simulink model "arducopter"  (R2024b)
settings: Solver=FixedStepAuto  StartTime=0.0  StopTime=simIn.param.timeEnd  FixedStep=simIn.param.dt  RelTol=1e-3
undefined symbols (not defined in the file or in its folder): DiscIntNeverNeededParam, sim, simIn
libraries: simulink x60, slident x4, vrlib x1
(part 1 of 9)
settings Model: Creator=f02brede  LastModifiedBy=I012407
settings SolverCC: AlgebraicLoopSolver=TrustRegion
settings OptimizationCC: BlockReduction=off  DefaultParameterBehavior=Inlined  BufferReuse=off
settings DebuggingCC: ParamSuppressDoubleToSinglePrecisionLossMsg=on  UnconnectedInputMsg=warning  UnconnectedOutputMsg=warning  UnconnectedLineMsg=warning  UnderSpecifiedDimensionMsg=warning
settings ModelReferenceCC: EnableRefExpFcnMdlSchedulingChecks=on
settings RTWCC: GPUComputeCapability=3.5  DLArmComputeVersion=19.05

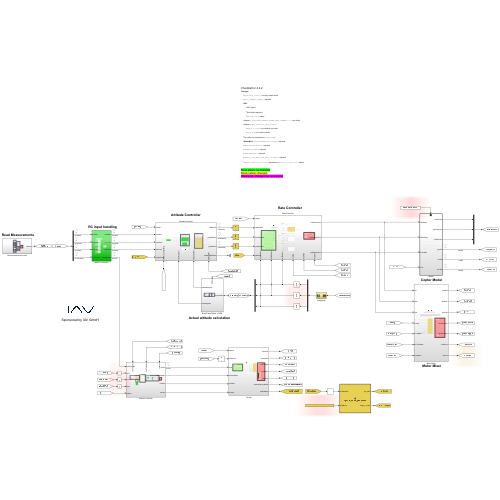
[thumbnail: Simulink's stored preview of the top-level diagram]
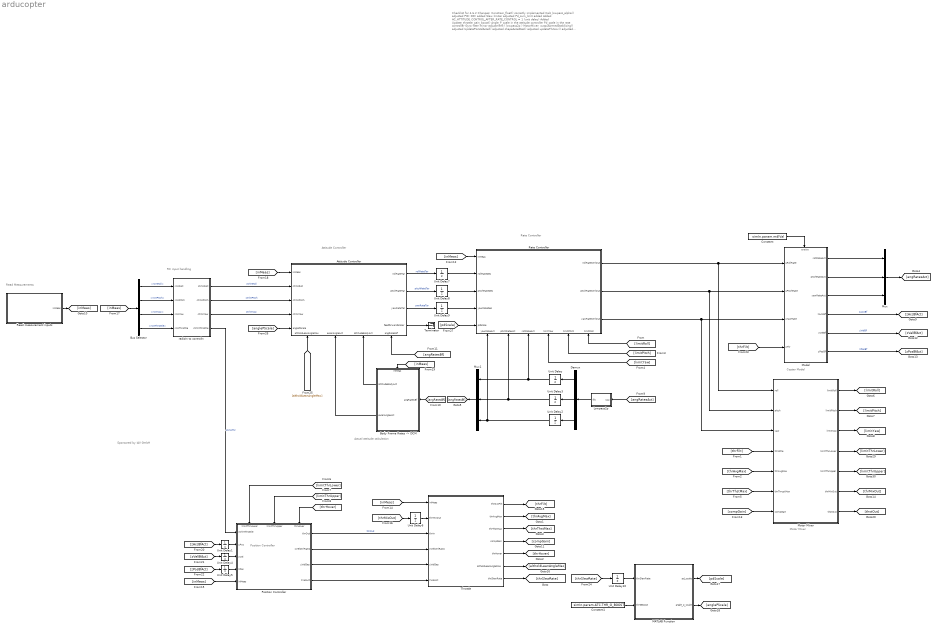
== system arducopter ==
  note: Checklist for 4.6.2
      | Changes:
      | Constrain_float() correctly implemented
      | Calc_lowpass_alpha() adjusted
      | PID: DFF added
      | Slew limiter adjusted
      | Pd_sum_limit added
      |
      | Added AC_ATTITUDE_CONTROL_AFTER_RATE_CONTROL = 1 (unit delay)
      | Added Update_throttle_gain_boost() Angle_P_scale in the attitude controller
      | Pd_scale in the rate controller
      |
      | Gyro filter minor adjustment ( lowpass2p )
      | MotorMixer: outputArmedStabilizing() adjusted
      | UpdatePosVelAccel() adjusted
      | shapeAccelDes() adjusted
      | updateThrHov() adjusted
      | Update_lift_max_from_batt_voltage() adjusted
      | Update_throttle_filter() adjusted and throttle_slew_filter added
      |
      | Bock green: no changes
      | Block yellow: changes
      | Block pink: changes but no solution
  note: Read Measurements
  note: RC input handling
  note: Attitude Controller
  note: Position Controller
  note: Actual attitude calculation
  note: Rate Controller
  note: Copter Model
  note: Motor Mixer
  note: Sponsored by IAV GmbH
  Attitude Controller : Subsystem
      settings: PortSchema="{\"entries\":[{\"content\":{\"sides\":[{\"content\":{\"connectorIds\":[\"In1\",\"In2\",\"In3\",\"In4\",\"In5\"]},\"type\":\"ConnectorPlacement.EquallySpacedRectSide\",\"uuid\":\"be329309-f60f-4247-8f12-99293f1f15e2\"},{\"content\":{\"connectorIds\":[\"Out1\",\"Out2\",\"Out3\",\"Out4\"],\"side\":\"RIGHT\"},\"type\":\"ConnectorPlacement.EquallySpacedRectSide\",\"uuid\":\"c2d00d61-d122-496e-b903-ccd22f2a218f\"},{\"content\":{\"side\":\"TOP\"},\"type\":\"ConnectorPlacement.EquallySpacedRectSide\",\"uuid\":\"754e14e5-9744-47de-9a4b-82f23abee3a3\"},{\"content\":{\"connectorIds\":[\"In6\",\"In7\",\"In8\",\"In9\"],\"side\":\"BOTTOM\"},\"type\":\"ConnectorPlacement.EquallySpacedRectSide\",\"uuid\":\"be89750d-8e93-4dd5-898c-e5776ff84547\"}]},\"type\":\"ConnectorPlacement.EquallySpacedConnector\",\"uuid\":\"7867ed09-773f-4285-9280-958eb598c3c9\"}],\"packageUris\":[\"http://schema.mathworks.com/mf0/Connector/R2020b\"],\"version\":\"1.0\"}"
  "Body Frame Rates -> DCM" : Subsystem
      settings: PortSchema="{\"entries\":[{\"content\":{\"sides\":[{\"content\":{\"connectorIds\":[\"In1\"]},\"type\":\"ConnectorPlacement.EquallySpacedRectSide\",\"uuid\":\"b5a1df0d-dabf-40be-945b-766674ab7f8a\"},{\"content\":{\"connectorIds\":[\"Out1\",\"Out2\"],\"side\":\"RIGHT\"},\"type\":\"ConnectorPlacement.EquallySpacedRectSide\",\"uuid\":\"df9d5bb2-532d-49d7-bb71-db77180d8edc\"},{\"content\":{\"connectorIds\":[\"In2\"],\"side\":\"TOP\"},\"type\":\"ConnectorPlacement.EquallySpacedRectSide\",\"uuid\":\"d376726d-d96e-422a-81b7-0e4338bb2c38\"}]},\"type\":\"ConnectorPlacement.EquallySpacedConnector\",\"uuid\":\"2a47101d-f111-46e9-ab13-8c5a8aa6bb71\"}],\"packageUris\":[\"http://schema.mathworks.com/mf0/Connector/R2020b\"],\"version\":\"1.0\"}"
  Bus Selector : BusSelector  OutputSignals=RCIN.rcinRoll,RCIN.rcinPitch,RCIN.rcinYaw,RCIN.rcinThrottle
  Constant : Constant  Value=simIn.param.mdlVal
  Constant1 : Constant  Value=simIn.param.ATC.THR_G_BOOST
  Demux : Demux  Outputs=3
  Lowpass2p : Subsystem
  MATLAB Function : MATLAB Function  TreatAsAtomicUnit=on
  Model : Subsystem
  Motor Mixer : Subsystem
  Mux : Mux  Inputs=3
  Mux1 : Mux  Inputs=3
  Position Controller : Subsystem
      settings: PortSchema="{\"entries\":[{\"content\":{\"sides\":[{\"content\":{\"connectorIds\":[\"In1\",\"In2\",\"In3\",\"In4\",\"In5\"]},\"type\":\"ConnectorPlacement.EquallySpacedRectSide\",\"uuid\":\"373ae21e-4a6c-4b99-84f1-ac5f8a8ac7e4\"},{\"content\":{\"connectorIds\":[\"Out1\",\"Out2\",\"Out3\",\"Out4\"],\"side\":\"RIGHT\"},\"type\":\"ConnectorPlacement.EquallySpacedRectSide\",\"uuid\":\"b87000f3-0870-478f-96d5-bf9fbf48201f\"},{\"content\":{\"connectorIds\":[\"In6\",\"In7\",\"In8\"],\"side\":\"TOP\"},\"type\":\"ConnectorPlacement.EquallySpacedRectSide\",\"uuid\":\"fdc4322a-c616-417b-b4c1-4fa4efa7a345\"}]},\"type\":\"ConnectorPlacement.EquallySpacedConnector\",\"uuid\":\"66c5051f-cbed-470e-8eb0-2aea9e9650fc\"}],\"packageUris\":[\"http://schema.mathworks.com/mf0/Connector/R2020b\"],\"version\":\"1.0\"}"
  Rate Controller : Subsystem
      settings: PortSchema="{\"entries\":[{\"content\":{\"sides\":[{\"content\":{\"connectorIds\":[\"In1\",\"In2\",\"In3\",\"In4\",\"In5\"]},\"type\":\"ConnectorPlacement.EquallySpacedRectSide\",\"uuid\":\"8a701ca7-ce38-496e-9f89-73a8426d5a34\"},{\"content\":{\"connectorIds\":[\"Out1\",\"Out2\",\"Out3\"],\"side\":\"RIGHT\"},\"type\":\"ConnectorPlacement.EquallySpacedRectSide\",\"uuid\":\"363a0e2e-6acc-4f21-9121-ba7c8748d9b4\"},{\"content\":{\"side\":\"TOP\"},\"type\":\"ConnectorPlacement.EquallySpacedRectSide\",\"uuid\":\"4d7a2121-90ee-4dbe-91e3-b86ad0b96fd9\"},{\"content\":{\"connectorIds\":[\"In6\",\"In7\",\"In8\",\"In9\",\"In10\",\"In11\"],\"side\":\"BOTTOM\"},\"type\":\"ConnectorPlacement.EquallySpacedRectSide\",\"uuid\":\"495eef18-c57e-4f49-baa4-5500712935f3\"}]},\"type\":\"ConnectorPlacement.EquallySpacedConnector\",\"uuid\":\"9c8722b4-18d5-4647-94e4-af7446d3f664\"}],\"packageUris\":[\"http://schema.mathworks.com/mf0/Connector/R2020b\"],\"version\":\"1.0\"}"
  Read measurement inputs : Subsystem
  Terminator : Terminator
  Throttle : Subsystem
  Unit Delay{,2,6..10} (7 alike) : UnitDelay  SampleTime=-1  HasFrameUpgradeWarning=on
  Unit Delay1 : UnitDelay  InitialCondition=simIn.init.PSCD.accAct  SampleTime=-1  HasFrameUpgradeWarning=on
  Unit Delay3 : UnitDelay  InitialCondition=simIn.models.PitchInit  SampleTime=-1  HasFrameUpgradeWarning=on
  Unit Delay4 : UnitDelay  InitialCondition=simIn.init.PSCD.velAct  SampleTime=-1  HasFrameUpgradeWarning=on
  Unit Delay5 : UnitDelay  InitialCondition=simIn.init.PSCD.posAct  SampleTime=-1  HasFrameUpgradeWarning=on
  radioIn to controlIn : Subsystem
  wires:
  [compGain] -> Motor Mixer/7(compGain)
  Rate Controller/3(yawRateCtrlOut) -> Model/3(uYawRate), Motor Mixer/3(yaw)
  Motor Mixer/5(limitThrUpper) -> [limitThrUpper]
  [thrThstMax] -> Motor Mixer/6(thrThrustMax)
  Motor Mixer/4(limitThrLower) -> [limitThrLower]
  Motor Mixer/7(thstOut) -> [thstOut]
  Motor Mixer/2(limitPitch) -> [limitPitch]
  Motor Mixer/3(limitYaw) -> [limitYaw]
  Motor Mixer/6(thrMixOut) -> [thrMixOut]
  [thrFilt] -> Motor Mixer/4(throttle)
  [thrAvgMax] -> Motor Mixer/5(thrAvgMax)
  Motor Mixer/1(limitRoll) -> [limitRoll]
  Throttle/2(thrAvgMax) -> [thrAvgMax]
  Throttle/3(thrThstMax) -> [thrThstMax]
  Throttle/4(compGain) -> [compGain]
  [limitYaw] -> Rate Controller/9(limitYaw)
  [limitPitch] -> Rate Controller/10(limitPitch)
  [limitRoll] -> Rate Controller/11(limitRoll)
  Throttle/5(thrHover) -> [thrHover]
  [limitThrLower] -> Position Controller/6(limitThrLower)
  [limitThrUpper] -> Position Controller/7(limitThrUpper)
  Position Controller/1(thrOut) -> Throttle/3(thrIn)  "thrOut"
  Position Controller/2(zVelCtrlRatio) -> Throttle/4(zVelCtrlRatio)
  Position Controller/3(zVelDes) -> Throttle/5(zVelDes)
  Position Controller/4(zVelAct) -> Throttle/6(zVelAct)
  Model/1(rollRateAct) -> Mux/1
  Model/2(pitchRateAct) -> Mux/2
  Model/3(yawRateAct) -> Mux/3
  Unit Delay/1 -> Mux1/1, Rate Controller/8(rollRateAct)
  Unit Delay2/1 -> Mux1/3, Rate Controller/6(yawRateAct)
  Read measurement inputs/1(inMeas) -> [inMeas]
  [inMeas] -> Rate Controller/1(inMeas)
  [inMeas] -> Throttle/1(inMeas)
  [inMeas] -> Position Controller/5(inMeas)
  [inMeas] -> Bus Selector/1
  Demux/2 -> Unit Delay3/1
  Mux/1 -> [angRatesAct]
  Demux/1 -> Unit Delay/1
  Demux/3 -> Unit Delay2/1
  [angRatesAct] -> Lowpass2p/1(raw)
  Lowpass2p/1(filt) -> Demux/1
  Unit Delay3/1 -> Mux1/2, Rate Controller/7(pitchRateAct)
  Rate Controller/2(pitchRateCtrlOut) -> Motor Mixer/2(pitch), Model/2(uPitchRate)
  Rate Controller/1(rollRateCtrlOut) -> Motor Mixer/1(roll), Model/1(uRollRate)
  Attitude Controller/2(pitchRateTar) -> Unit Delay8/1  "pitchRateTar"
  Attitude Controller/3(yawRateTar) -> Unit Delay9/1  "yawRateTar"
  Bus Selector/1 -> radioIn to controlIn/1(rcInRoll)  "<rcinRoll>"
  Bus Selector/2 -> radioIn to controlIn/2(rcInPitch)  "<rcinPitch>"
  Bus Selector/3 -> radioIn to controlIn/3(rcInYaw)  "<rcinYaw>"
  "Body Frame Rates -> DCM"/1(attitudeBodyAct) -> Attitude Controller/8(attitudeBodyAct)
  Mux1/1 -> [angRatesBf]
  [angRatesBf] -> "Body Frame Rates -> DCM"/1(angRatesBf)
  [angRatesBf] -> Attitude Controller/9(angRatesBf)
  [inMeas] -> Attitude Controller/1(inMeas)
  Attitude Controller/4(feedforwardScaler) -> Terminator/1
  [inMeas] -> "Body Frame Rates -> DCM"/2(inMeas)
  radioIn to controlIn/1(ctrlInRoll) -> Attitude Controller/2(ctrlInRoll)  "ctrlInRoll"
  radioIn to controlIn/2(ctrlInPitch) -> Attitude Controller/3(ctrlInPitch)  "ctrlInPitch"
  radioIn to controlIn/3(ctrlInYaw) -> Attitude Controller/4(ctrlInYaw)  "ctrlInYaw"
  Attitude Controller/1(rollRateTar) -> Unit Delay7/1  "rollRateTar"
  Constant/1 -> Model/Enable
  "Body Frame Rates -> DCM"/2(eulerAngleAct) -> Attitude Controller/7(eulerAngleAct)
  Model/4(zAccBf) -> [zAccBfAct]  "zAccBf"
  [thrFilt] -> Model/4(uThr)
  Model/5(zVelBf) -> [zVelBfAct]  "zVelBf"
  Model/6(zPosBf) -> [zPosBfAct]  "zPosBf"
  [zAccBfAct] -> Unit Delay1/1
  [zVelBfAct] -> Unit Delay4/1
  [zPosBfAct] -> Unit Delay5/1
  [thrHover] -> Position Controller/8(thrHover)
  Unit Delay1/1 -> Position Controller/2(zAcc)
  Unit Delay4/1 -> Position Controller/3(zVel)
  Unit Delay5/1 -> Position Controller/4(zPos)
  Bus Selector/4 -> radioIn to controlIn/4(rcInThrottle)  "<rcinThrottle>"
  radioIn to controlIn/4(ctrlInThrottle) -> Position Controller/1(ctrlInThrottle)  "ctrlInThr"
  Throttle/1(thrOutFilt) -> [thrFilt]
  [thrMixOut] -> Unit Delay6/1
  Unit Delay6/1 -> Throttle/2(thrMixOut)
  [altholdLeanAngleMax] -> Attitude Controller/6(altholdLeanAngleMax)
  Throttle/6(altholdLeanAngleMax) -> [altholdLeanAngleMax]
  Unit Delay9/1 -> Rate Controller/4(yawRateDes)
  Unit Delay8/1 -> Rate Controller/3(pitchRateDes)
  Unit Delay7/1 -> Rate Controller/2(rollRateDes)
  Throttle/7(thrSlewRate) -> [thrSlewRate]
  Constant1/1 -> MATLAB Function/2(thrGBoost)
  [thrSlewRate] -> Unit Delay10/1
  MATLAB Function/1(pd_scale) -> [pdScale]
  MATLAB Function/2(angle_p_scale) -> [anglePScale]
  [anglePScale] -> Attitude Controller/5(anglePScale)
  [pdScale] -> Rate Controller/5(pdScale)
  Unit Delay10/1 -> MATLAB Function/1(thrSlewRate)

== system arducopter/Attitude Controller ==
  note: input_euler_angle_roll_pitch_euler_rate_yaw() & attitude_controller_run_quat()
      | Calculation of target euler rates and angles and angular velocities
  note: Mode::get_pilot_desired_lean_angles() & Mode::get_pilot_desired_yaw_rate()
      | Conversion from raw pilot inputs to desired roll and pitch angles and yaw rate
  note: Determines the angleLimit (angle_limit_cd) based on the flight mode
  note: Sponsored by IAV GmbH
  inMeas : Inport
  ctrlInRoll : Inport  Port=2
  ctrlInPitch : Inport  Port=3
  ctrlInYaw : Inport  Port=4
  anglePScale : Inport  Port=5
  altholdLeanAngleMax : Inport  Port=6
  eulerAngleAct : Inport  Port=7
  attitudeBodyAct : Inport  Port=8
  angRatesBf : Inport  Port=9
  Bus Selector : BusSelector  OutputSignals=CTUN.thrInMeas
  Constant : Constant  Value=simIn.param.ANGLE_MAX
  Constant1 : Constant  Value=simIn.param.PILOT_Y_EXPO
  Constant2 : Constant  Value=simIn.param.PILOT_Y_RATE
  Constant3 : Constant  Value=simIn.param.RCIN.ROLL_PITCH_YAW_INPUT_MAX
  Demux : Demux  Outputs=3
  Determine angleLimit : Subsystem
  MATLAB Function : MATLAB Function  TreatAsAtomicUnit=on
  MATLAB Function1 : MATLAB Function  TreatAsAtomicUnit=on
  cdeg to radians : Gain  Gain=0.01*pi/180
  cdeg to radians1 : Gain  Gain=0.01*pi/180
  cdeg/s to radians/s : Gain  Gain=0.01*pi/180
  input_euler_angle_roll_pitch_euler_rate_yaw() : Subsystem
      settings: PortSchema="{\"entries\":[{\"content\":{\"sides\":[{\"content\":{\"connectorIds\":[\"In1\",\"In2\",\"In3\",\"In4\",\"In5\",\"In6\"]},\"type\":\"ConnectorPlacement.EquallySpacedRectSide\",\"uuid\":\"a7f2758f-6981-4691-a616-9de398d31e49\"},{\"content\":{\"connectorIds\":[\"Out1\",\"Out2\"],\"side\":\"RIGHT\"},\"type\":\"ConnectorPlacement.EquallySpacedRectSide\",\"uuid\":\"ab82c46a-21a0-4466-8d5f-7cb35c1d2ba7\"},{\"content\":{\"connectorIds\":[\"In7\",\"In8\"],\"side\":\"TOP\"},\"type\":\"ConnectorPlacement.EquallySpacedRectSide\",\"uuid\":\"f47afcce-c5f7-4588-aa52-961f89e87fe1\"}]},\"type\":\"ConnectorPlacement.EquallySpacedConnector\",\"uuid\":\"c65a3016-6632-4380-919e-0448495ac13d\"}],\"packageUris\":[\"http://schema.mathworks.com/mf0/Connector/R2020b\"],\"version\":\"1.0\"}"
  rollRateTar : Outport
  pitchRateTar : Outport  Port=2
  yawRateTar : Outport  Port=3
  feedforwardScaler : Outport  Port=4
  wires:
  ctrlInRoll/1 -> MATLAB Function/1(rollIn)
  ctrlInPitch/1 -> MATLAB Function/2(pitchIn)
  Constant/1 -> MATLAB Function/3(angleMax)
  Constant1/1 -> MATLAB Function1/2(pilotYawExpo)
  Constant2/1 -> MATLAB Function1/3(pilotYawRate)
  MATLAB Function/1(rollOut) -> cdeg to radians/1
  MATLAB Function/2(pitchOut) -> cdeg to radians1/1
  cdeg to radians/1 -> input_euler_angle_roll_pitch_euler_rate_yaw()/1(rollAngDes)  "rollLeanAngleDes"
  cdeg to radians1/1 -> input_euler_angle_roll_pitch_euler_rate_yaw()/2(pitchAngDes)  "pitchLeanAngleDes"
  attitudeBodyAct/1 -> input_euler_angle_roll_pitch_euler_rate_yaw()/5(attitudeBodyAct)
  angRatesBf/1 -> input_euler_angle_roll_pitch_euler_rate_yaw()/6(angRatesBf)
  Demux/2 -> pitchRateTar/1
  Demux/1 -> rollRateTar/1
  Demux/3 -> yawRateTar/1
  input_euler_angle_roll_pitch_euler_rate_yaw()/1(angVelBodyTarget) -> Demux/1  "angVelBody"
  input_euler_angle_roll_pitch_euler_rate_yaw()/2(feedforwardScaler) -> feedforwardScaler/1
  inMeas/1 -> Bus Selector/1
  Bus Selector/1 -> [throttle]  "<thrInMeas>"
  [throttle] -> input_euler_angle_roll_pitch_euler_rate_yaw()/7(throttle)
  eulerAngleAct/1 -> input_euler_angle_roll_pitch_euler_rate_yaw()/4(eulerAngleAct)
  ctrlInYaw/1 -> MATLAB Function1/1(yawIn)
  Constant3/1 -> MATLAB Function/5(rpyInputMax)
  cdeg/s to radians/s/1 -> input_euler_angle_roll_pitch_euler_rate_yaw()/3(yawRateDes)  "yawRateDes"
  MATLAB Function1/1(yawOut) -> cdeg/s to radians/s/1  "yawRateDes"
  altholdLeanAngleMax/1 -> Determine angleLimit/1(altholdLeanAngleMax)
  Determine angleLimit/1(angleLimit) -> MATLAB Function/4(angleLimit)
  anglePScale/1 -> input_euler_angle_roll_pitch_euler_rate_yaw()/8(anglePScale)

== system arducopter/Body Frame Rates -> DCM ==
  note: QuaternionT<T>::from_rotation_matrix()
      | Calculation of the quaternion of the body-frame attitude.
      | Function is called in AC_AttitudeControl::attitude_controller_run_quat() -> AP_AHRS::get_quat_body_to_ned()
  note: The resulting matrix is updated in AP_AHRS_View::update(). There, it is rotated by the rotation matrix of the view, which is created in the constructor of AP_AHRS_View. For a copter, it is zero (see system.cpp: ahrs_view = ahrs.create_view(ROTATION_NONE))
      |
      | The resulting matrix represents the rotation matrix that is used to calculate the "measured" angles of the ATT message.
  note: $\Delta \underline{\underline{R}} = \underline{\underline{R}} \, \Delta \underline{\underline{w}}$
  note: Taken from Matrix3<T>::rotate() in matrix.cpp
  note: Source: https://academicflight.com/articles/kinematics/rotation-formalisms/rotation-matrix/
  note: Create cross-product equivalent matrix of vector
  note: Source: AP_AHRS_DCM::matrix_update() and Matrix3<T>::rotate()
      | - Corrections for gyro drifts (_omega_I, _omega_P, _omega_yaw_P) were left out.
  note: Update DCM matrix
  note: $\Delta \underline{\underline{w}} = \underline{\underline{\omega}} \, T_s$
  note: $\underline{\underline{R}}_{\, \mathrm{k}} = \Delta \underline{\underline{R}} + \underline{\underline{R}}_{\, \mathrm{k-1}}$
  note: Calculation of _body_dcm_matrix aka rot_body_to_ned
  note: Correction of DCM by difference between controller and body
      | frames.
      | Taken from AP_AHRS_DCM::euler_angles()
  note: Sponsored by IAV GmbH
  angRatesBf : Inport
  inMeas : Inport  Port=2
  BF2FC : Constant  Value=simIn.param.AHRS.BF2FC
  Bus Selector : BusSelector  OutputSignals=ATT.rollAngleActMeas,ATT.pitchAngleActMeas,ATT.yawAngleActMeas
  Bus Selector1 : BusSelector  OutputSignals=ATT.rollAngleActMeas,ATT.pitchAngleActMeas,ATT.yawAngleActMeas
  Constant : Constant  Value=0  OutDataTypeStr=single
  Constant1 : Constant  Value=simIn.param.attCtrlVal
  Constant4 : Constant  Value=simIn.param.attCtrlVal
  Data Type Conversion : DataTypeConversion  OutDataTypeStr=single  SaturateOnIntegerOverflow=off  RndMeth=Floor
  Data Type Conversion1 : DataTypeConversion  OutDataTypeStr=single  SaturateOnIntegerOverflow=off  RndMeth=Floor
  Gain2 : Gain  Gain=simIn.param.dt  OutDataTypeStr=single
  Gain3 : Gain  Gain=[1 1 -1]
  Gain4 : Gain  Gain=[-1 1 1]
  Gain5 : Gain  Gain=[1 -1 1]
  MATLAB Function : MATLAB Function  TreatAsAtomicUnit=on
  MATLAB Function1 : MATLAB Function  TreatAsAtomicUnit=on
  MATLAB Function2 : MATLAB Function  TreatAsAtomicUnit=on
  MATLAB Function3 : MATLAB Function  TreatAsAtomicUnit=on
  Matrix Concatenate : Concatenate  NumInputs=3  Mode=Multidimensional array  ConcatenateDimension=2
  Mux : Mux  Inputs=3
  Mux1 : Mux  Inputs=3
  Product : Product  Multiplication=Matrix(*)
  Product1 : Product  Multiplication=Matrix(*)
  Selector : Selector  InputPortWidth=4  IndexOptions=Index vector (dialog)  Indices=[1 4 3]  OutputSizes=1
  Selector1 : Selector  InputPortWidth=4  IndexOptions=Index vector (dialog)  Indices=[4 1 2]  OutputSizes=1
  Selector2 : Selector  InputPortWidth=4  IndexOptions=Index vector (dialog)  Indices=[3 2 1]  OutputSizes=1
  Sum : Sum  Inputs=++|
  Switch : Switch  Criteria=u2 > Threshold  SaturateOnIntegerOverflow=off  InputSameDT=off
  Switch1 : Switch  Criteria=u2 > Threshold  SaturateOnIntegerOverflow=off  InputSameDT=off
  Unit Delay : UnitDelay  InitialCondition=simIn.init.ATT.DCM  SampleTime=-1  HasFrameUpgradeWarning=on
  Vector Concatenate : Concatenate
  attitudeBodyAct : Outport
  eulerAngleAct : Outport  Port=2
  wires:
  angRatesBf/1 -> Vector Concatenate/2
  Vector Concatenate/1 -> Selector/1, Selector1/1, Selector2/1
  Selector/1 -> Gain3/1
  Constant/1 -> Vector Concatenate/1
  Selector2/1 -> Gain5/1
  Selector1/1 -> Gain4/1
  Gain3/1 -> Matrix Concatenate/1
  Gain4/1 -> Matrix Concatenate/2
  Gain5/1 -> Matrix Concatenate/3
  Matrix Concatenate/1 -> Gain2/1
  Unit Delay/1 -> Product/1, Sum/1
  Product/1 -> Sum/2
  Sum/1 -> Product1/1, Unit Delay/1  "DCM"
  Gain2/1 -> Product/2
  BF2FC/1 -> Product1/2
  Product1/1 -> MATLAB Function1/1(rotMat), MATLAB Function/1(dcm)  "bodyDCM"
  MATLAB Function/1(quaternion) -> Data Type Conversion/1
  [meas] -> Bus Selector/1
  Bus Selector/2 -> MATLAB Function2/2(pitch)  "<pitchAngleActMeas>"
  Bus Selector/1 -> MATLAB Function2/1(roll)  "<rollAngleActMeas>"
  Bus Selector/3 -> MATLAB Function2/3(yaw)  "<yawAngleActMeas>"
  MATLAB Function3/1(quaternion) -> Data Type Conversion1/1
  MATLAB Function2/1(rotMat) -> MATLAB Function3/1(dcm)  "bodyDCMMeas"
  MATLAB Function1/1(roll) -> Mux/1  "rollAngleAct"
  MATLAB Function1/2(pitch) -> Mux/2  "pitchAngleAct"
  MATLAB Function1/3(yaw) -> Mux/3  "yawAngleAct"
  Switch/1 -> attitudeBodyAct/1
  Data Type Conversion1/1 -> Switch/1
  Data Type Conversion/1 -> Switch/3
  Constant4/1 -> Switch/2
  Switch1/1 -> eulerAngleAct/1
  Constant1/1 -> Switch1/2
  Mux/1 -> Switch1/3
  inMeas/1 -> [meas]
  [meas] -> Bus Selector1/1
  Bus Selector1/1 -> Mux1/1  "<rollAngleActMeas>"
  Bus Selector1/2 -> Mux1/2  "<pitchAngleActMeas>"
  Bus Selector1/3 -> Mux1/3  "<yawAngleActMeas>"
  Mux1/1 -> Switch1/1

== system arducopter/Lowpass2p ==
  raw : Inport
  Constant : Constant  Value=simIn.param.INS.GYRO_FILTER
  Constant1 : Constant  Value=simIn.param.INS.GYRO_RATE
  Demux : Demux  Outputs=3
  Lowpass Pitch : Subsystem
  Lowpass Roll : Subsystem
  Lowpass Yaw : Subsystem
  Mux : Mux  Inputs=3
  filt : Outport
  wires:
  raw/1 -> Demux/1
  Demux/1 -> [rollRaw]
  Demux/3 -> [yawRaw]
  Demux/2 -> [pitchRaw]
  [rollRaw] -> Lowpass Roll/1(sample)
  [pitchRaw] -> Lowpass Pitch/1(sample)
  [yawRaw] -> Lowpass Yaw/1(sample)
  Mux/1 -> filt/1
  Lowpass Roll/1(y) -> [rollFilt]
  Lowpass Pitch/1(y) -> [pitchFilt]
  Lowpass Yaw/1(y) -> [yawFilt]
  [rollFilt] -> Mux/1
  [pitchFilt] -> Mux/2
  [yawFilt] -> Mux/3
  Constant/1 -> [cutoffFreq]
  Constant1/1 -> [sampleFreq]
  [sampleFreq] -> Lowpass Roll/2(sampleFreq)
  [cutoffFreq] -> Lowpass Roll/3(cutoffFreq)
  [cutoffFreq] -> Lowpass Pitch/3(cutoffFreq)
  [sampleFreq] -> Lowpass Pitch/2(sampleFreq)
  [sampleFreq] -> Lowpass Yaw/2(sampleFreq)
  [cutoffFreq] -> Lowpass Yaw/3(cutoffFreq)

== system arducopter/Model ==
  uRollRate : Inport
  uPitchRate : Inport  Port=2
  uYawRate : Inport  Port=3
  uThr : Inport  Port=4
  Enable : EnablePort
  Constant : Constant  Value=simIn.models.VerticalInInit
  Data Type Conversion{,2..3,6} (4 alike) : DataTypeConversion  OutDataTypeStr=double  SaturateOnIntegerOverflow=off  RndMeth=Floor
  Data Type Conversion{1,4..5,7} (4 alike) : DataTypeConversion  OutDataTypeStr=single  SaturateOnIntegerOverflow=off  RndMeth=Floor
  Discrete-Time Integrator : DiscreteIntegrator  InitialCondition=simIn.init.PSCD.velAct  SampleTime=0.0025  ICPrevOutput=DiscIntNeverNeededParam  ICPrevScaledInput=DiscIntNeverNeededParam
  Discrete-Time Integrator1 : DiscreteIntegrator  InitialCondition=simIn.init.PSCD.posAct  SampleTime=-1  ICPrevOutput=DiscIntNeverNeededParam  ICPrevScaledInput=DiscIntNeverNeededParam
  Idmodel : slident/Models/Idmodel  sys=simIn.models.PitchAxis  IC=simIn.models.PitchInit  noi=off  seed=[]
  Idmodel1 : slident/Models/Idmodel  sys=simIn.models.RollAxis  IC=simIn.models.RollInit  noi=off  seed=[]
  Idmodel2 : slident/Models/Idmodel  sys=simIn.models.YawAxis  IC=simIn.models.YawInit  noi=off  seed=[]
  Idmodel3 : slident/Models/Idmodel  sys=simIn.models.VerticalAxis  IC=0  noi=off  seed=[]
  Sum : Sum  Inputs=|+-
  rollRateAct : Outport
  pitchRateAct : Outport  Port=2
  yawRateAct : Outport  Port=3
  zAccBf : Outport  Port=4
  zVelBf : Outport  Port=5
  zPosBf : Outport  Port=6
  wires:
  uPitchRate/1 -> Data Type Conversion/1
  uYawRate/1 -> Data Type Conversion2/1
  Idmodel1/1 -> Data Type Conversion4/1
  uRollRate/1 -> Data Type Conversion3/1
  Idmodel2/1 -> Data Type Conversion5/1
  Data Type Conversion/1 -> Idmodel/1
  Data Type Conversion2/1 -> Idmodel2/1
  Data Type Conversion3/1 -> Idmodel1/1
  Data Type Conversion4/1 -> rollRateAct/1
  Data Type Conversion1/1 -> pitchRateAct/1
  Data Type Conversion5/1 -> yawRateAct/1
  Idmodel/1 -> Data Type Conversion1/1
  Data Type Conversion6/1 -> Idmodel3/1
  Idmodel3/1 -> Data Type Conversion7/1
  Sum/1 -> Data Type Conversion6/1
  uThr/1 -> Sum/1
  Data Type Conversion7/1 -> Discrete-Time Integrator/1, zAccBf/1
  Constant/1 -> Sum/2
  Discrete-Time Integrator/1 -> Discrete-Time Integrator1/1, zVelBf/1
  Discrete-Time Integrator1/1 -> zPosBf/1

== system arducopter/Motor Mixer ==
  note: Motor Mixer Output
  note: This function calculates the outputs to the motors based on the requested roll, pitch, yaw and throttle thrust. At first, the maximum allowed yaw is calculated. On the basis of the difference between the maximum and minimum value of the combined roll, pitch and yaw thrust of the motors, the thrust values are scaled within the valid output range. The final motor commands are calculated by the sum of the combined roll, pitch and yaw thrust and and the demanded throttle thrust, which might be set to a lower value when the combined thrust demand of roll, pitch and yaw exceed the possbile thrust.
  note: Motor Mixer - Calculation of outputs to motors.
  note: Sponsored by IAV GmbH
  roll : Inport
  pitch : Inport  Port=2
  yaw : Inport  Port=3
  throttle : Inport  Port=4
  thrAvgMax : Inport  Port=5
  thrThrustMax : Inport  Port=6
  compGain : Inport  Port=7
  Calculate motor thrust : MATLAB Function  TreatAsAtomicUnit=on
  Clock : Clock
  Constant : Constant  Value=simIn.param.NUM_MOTORS
  Constant1 : Constant  Value=simIn.param.AXIS_FAC_MOTORS.pitch  VectorParams1D=off
  Constant11 : Constant  Value=simIn.param.MOT.YAW_HEADROOM
  Constant12 : Constant  Value=simIn.param.AXIS_FAC_MOTORS.throttle  VectorParams1D=off
  Constant2 : Constant  Value=simIn.param.AXIS_FAC_MOTORS.roll  VectorParams1D=off
  Constant3 : Constant  Value=simIn.param.AXIS_FAC_MOTORS.yaw  VectorParams1D=off
  Data Store Memory : DataStoreMemory  DataStoreName=thst_rpyt  ReadBeforeWriteMsg=warning  WriteAfterWriteMsg=warning  WriteAfterReadMsg=warning  InitialValue=zeros(simIn.param.NUM_MOTORS,1)  ShowAdditionalParam=off  OutDataTypeStr=single
  Data Type Conversion1 : DataTypeConversion  OutDataTypeStr=single  SaturateOnIntegerOverflow=off  RndMeth=Floor
  Data Type Conversion2 : DataTypeConversion  OutDataTypeStr=single  SaturateOnIntegerOverflow=off  RndMeth=Floor
  Terminator6 : Terminator
  ThrMixOutMeas : Lookup_n-D  NumberOfTableDimensions=1  BreakpointsForDimension1=simIn.signals.MOTQ.Time  Table=simIn.signals.MOTQ.ThrMixOut  InternalRulePriority=Speed  RndMeth=Simplest
  Vector Concatenate : Concatenate  NumInputs=4  Mode=Multidimensional array
  limitRoll : Outport
  limitPitch : Outport  Port=2
  limitYaw : Outport  Port=3
  limitThrLower : Outport  Port=4  SampleTime=simIn.param.dt
  limitThrUpper : Outport  Port=5  SampleTime=simIn.param.dt
  thrMixOut : Outport  Port=6
  thstOut : Outport  Port=7  SampleTime=simIn.param.dt
  wires:
  roll/1 -> Calculate motor thrust/1(roll)
  throttle/1 -> Calculate motor thrust/4(thrIn)
  Constant/1 -> Data Type Conversion1/1  "numMotors"
  Constant3/1 -> Vector Concatenate/3  "yaw_fac"
  Calculate motor thrust/1(limitRoll) -> limitRoll/1  "limitRoll"
  Calculate motor thrust/7(thstOut) -> thstOut/1  "thstOut"
  Constant2/1 -> Vector Concatenate/1  "roll_fac"
  Calculate motor thrust/2(limitPitch) -> limitPitch/1  "limitPitch"
  Vector Concatenate/1 -> Data Type Conversion2/1
  Constant11/1 -> Calculate motor thrust/8(yawHeadroom)
  Calculate motor thrust/6(thrOut) -> thrMixOut/1  "thrMixOut"
  Constant12/1 -> Vector Concatenate/4  "throttle_fac"
  Calculate motor thrust/3(limitYaw) -> limitYaw/1  "limitYaw"
  yaw/1 -> Calculate motor thrust/3(yaw)
  Constant1/1 -> Vector Concatenate/2  "pitch_fac"
  compGain/1 -> Calculate motor thrust/7(compGain)
  thrAvgMax/1 -> Calculate motor thrust/5(thrAvgMax)
  pitch/1 -> Calculate motor thrust/2(pitch)
  thrThrustMax/1 -> Calculate motor thrust/6(thrThstMaxIn)
  Data Type Conversion1/1 -> Calculate motor thrust/9(numMotors)
  Data Type Conversion2/1 -> Calculate motor thrust/10(facMotors)
  Calculate motor thrust/4(limitThrLower) -> limitThrLower/1  "limitThrLower"
  Calculate motor thrust/5(limitThrUpper) -> limitThrUpper/1  "limitThrUpper"
  ThrMixOutMeas/1 -> Terminator6/1  "thrMixOutMeas"
  Clock/1 -> ThrMixOutMeas/1

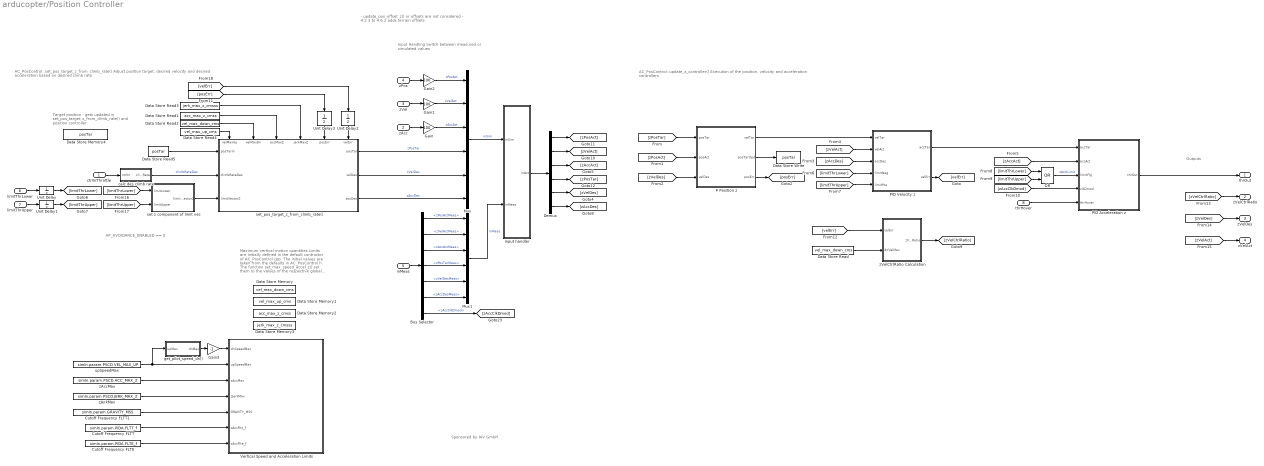
== system arducopter/Position Controller ==
  note: - update_pos_offset_z() or offsets are not considered
      | - 4.2.3 to 4.6.2 adds terrain offsets
  note: AP_AVOIDANCE_ENABLED == 0
  note: Input Handling
      | Switch between measured or simulated values
  note: Target position - gets updated in set_pos_target_z_from_climb_rate() and position controller
  note: Outputs
  note: Maximum vertical motion quantities
      | Limits are initially defined in the default contructor of AC_PosControl.cpp. The initial values are taken from the defaults in AC_PosControl.h. The function set_max_speed_accel_z() set them to the values of the respective global parameters.
  note: AC_PosControl::update_z_controller()
      | Execution of the position, velocity and acceleration controllers
  note: AC_PosControl::set_pos_target_z_from_climb_rate()
      | Adjust position target, desired velocity and desired acceleration based on desired climb rate
  note: Sponsored by IAV GmbH
  ctrlInThrottle : Inport
  zAcc : Inport  Port=2
  zVel : Inport  Port=3
  zPos : Inport  Port=4
  inMeas : Inport  Port=5
  limitThrLower : Inport  Port=6
  limitThrUpper : Inport  Port=7
  thrHover : Inport  Port=8
  Bus Selector : BusSelector  OutputSignals=PSCD.zPosActMeas,PSCD.zVelActMeas,PSCD.zAccActMeas,PSCD.zPosTarMeas,PSCD.zVelDesMeas,PSCD.zAccDesMeas,PIDA.zAccClkDmod
  Cutoff Frequency FLTE : Constant  Value=simIn.param.PIDA.FLTE_f
  Cutoff Frequency FLTT : Constant  Value=simIn.param.PIDA.FLTT_f
  Cutoff Frequency FLTT1 : Constant  Value=simIn.param.GRAVITY_MSS
  Data Store Memory : DataStoreMemory  DataStoreName=vel_max_down_cms  ReadBeforeWriteMsg=warning  WriteAfterWriteMsg=warning  WriteAfterReadMsg=warning  InitialValue=simIn.param.PSCD.VEL_MAX_DOWN_DFLT  ShowAdditionalParam=off  OutDataTypeStr=single
  Data Store Memory1 : DataStoreMemory  DataStoreName=vel_max_up_cms  ReadBeforeWriteMsg=warning  WriteAfterWriteMsg=warning  WriteAfterReadMsg=warning  InitialValue=simIn.param.PSCD.VEL_MAX_UP_DFLT  ShowAdditionalParam=off  OutDataTypeStr=single
  Data Store Memory2 : DataStoreMemory  DataStoreName=acc_max_z_cmss  ReadBeforeWriteMsg=warning  WriteAfterWriteMsg=warning  WriteAfterReadMsg=warning  InitialValue=simIn.param.PSCD.ACC_MAX_Z_DFLT  ShowAdditionalParam=off  OutDataTypeStr=single
  Data Store Memory3 : DataStoreMemory  DataStoreName=jerk_max_z_cmsss  ReadBeforeWriteMsg=warning  WriteAfterWriteMsg=warning  WriteAfterReadMsg=warning  InitialValue=simIn.param.PSCD.JERK_MAX_Z_DFLT  ShowAdditionalParam=off  OutDataTypeStr=single
  Data Store Memory4 : DataStoreMemory  DataStoreName=posTar  ReadBeforeWriteMsg=warning  WriteAfterWriteMsg=warning  WriteAfterReadMsg=warning  InitialValue=simIn.init.PIDA.posTar  ShowAdditionalParam=off  OutDataTypeStr=single
  Data Store Read : DataStoreRead  DataStoreName=vel_max_down_cms  IndexOptions=Index vector (dialog)  Indices=1  OutputSizes=1
  Data Store Read1 : DataStoreRead  DataStoreName=acc_max_z_cmss  IndexOptions=Index vector (dialog)  Indices=1  OutputSizes=1
  Data Store Read2 : DataStoreRead  DataStoreName=vel_max_down_cms  IndexOptions=Index vector (dialog)  Indices=1  OutputSizes=1
  Data Store Read3 : DataStoreRead  DataStoreName=jerk_max_z_cmsss  IndexOptions=Index vector (dialog)  Indices=1  OutputSizes=1
  Data Store Read4 : DataStoreRead  DataStoreName=vel_max_up_cms  IndexOptions=Index vector (dialog)  Indices=1  OutputSizes=1
  Data Store Read5 : DataStoreRead  DataStoreName=posTar  IndexOptions=Index vector (dialog)  Indices=1  OutputSizes=1
  Data Store Write : DataStoreWrite  DataStoreName=posTar  IndexOptions=Index vector (dialog)  Indices=1  OutputSizes=1
  Demux : Demux  Outputs=6
  Gain : Gain  Gain=100
  Gain1 : Gain  Gain=100
  Gain2 : Gain  Gain=100
  Gain3 : Gain  Gain=-1
  Mux : Mux  Inputs=6
  Mux1 : Mux  Inputs=6
  OR : Logic  Operator=OR  AllPortsSameDT=off  OutDataTypeStr=boolean
  P Position z : Subsystem
  PID Acceleration z : Subsystem
  PID Velocity z : Subsystem
  Unit Delay{,1..3} (4 alike) : UnitDelay  SampleTime=-1  HasFrameUpgradeWarning=on
  Vertical Speed and Acceleration Limits : MATLAB Function  TreatAsAtomicUnit=on
  calc des climb rate : Subsystem
  get_pilot_speed_dn() : Subsystem
  input handler : Subsystem
  set z component of limit vec : Subsystem
  set_pos_target_z_from_climb_rate() : Subsystem  SCDEnableBlockLinearizationSpecification=on
      settings: PortSchema="{\"entries\":[{\"content\":{\"sides\":[{\"content\":{\"connectorIds\":[\"In1\",\"In2\",\"In3\"]},\"type\":\"ConnectorPlacement.EquallySpacedRectSide\",\"uuid\":\"29e997f2-a41d-40eb-bc2d-84e38345938a\"},{\"content\":{\"connectorIds\":[\"Out1\",\"Out2\",\"Out3\"],\"side\":\"RIGHT\"},\"type\":\"ConnectorPlacement.EquallySpacedRectSide\",\"uuid\":\"a29b5bbc-9346-4610-a837-ea2075d679ab\"},{\"content\":{\"connectorIds\":[\"In4\",\"In5\",\"In6\",\"In7\",\"In8\",\"In9\"],\"side\":\"TOP\"},\"type\":\"ConnectorPlacement.EquallySpacedRectSide\",\"uuid\":\"7f9b6f9f-376d-46a1-a723-f63ba0f37065\"}]},\"type\":\"ConnectorPlacement.EquallySpacedConnector\",\"uuid\":\"aa147654-bb66-4ce5-98a1-f6a4b81869c5\"}],\"packageUris\":[\"http://schema.mathworks.com/mf0/Connector/R2020b\"],\"version\":\"1.0\"}"
  upSpeedMax : Constant  Value=simIn.param.PSCD.VEL_MAX_UP
  zAccMax : Constant  Value=simIn.param.PSCD.ACC_MAX_Z
  zJerkMax : Constant  Value=simIn.param.PSCD.JERK_MAX_Z
  zVelCtrlRatio Calculation : Subsystem
  thrOut : Outport
  zVelCtrlRatio : Outport  Port=2
  zVelDes : Outport  Port=3
  zVelAct : Outport  Port=4
  wires:
  [zPosTar] -> P Position z/1(posTar)
  [zPosAct] -> P Position z/2(posAct)
  P Position z/2(posTarUpd) -> Data Store Write/1
  [zVelDes] -> P Position z/3(velDes)
  P Position z/1(velTar) -> PID Velocity z/1(velTar)
  [zVelAct] -> PID Velocity z/2(velAct)
  [zAccDes] -> PID Velocity z/3(accDes)
  [limitThrLower] -> PID Velocity z/4(limitNeg)
  [limitThrUpper] -> PID Velocity z/5(limitPos)
  PID Velocity z/1(accTar) -> PID Acceleration z/1(accTar)
  [zAccAct] -> PID Acceleration z/2(accAct)
  [limitThrLower] -> OR/1
  [limitThrUpper] -> OR/2
  OR/1 -> PID Acceleration z/3(limitFlg)  "zAccILimit"
  PID Acceleration z/1(thrOut) -> thrOut/1
  [zAccClkDmod] -> PID Acceleration z/4(clkDmod)
  thrHover/1 -> PID Acceleration z/5(thrHover)
  limitThrUpper/1 -> Unit Delay1/1
  PID Velocity z/2(velErr) -> [velErr]
  [velErr] -> zVelCtrlRatio Calculation/1(velErr)
  Data Store Read/1 -> zVelCtrlRatio Calculation/2(dnVelMax)
  zVelCtrlRatio Calculation/1(zVelCtrlRatio) -> [zVelCtrlRatio]
  [zVelCtrlRatio] -> zVelCtrlRatio/1
  upSpeedMax/1 -> get_pilot_speed_dn()/1(upMax), Vertical Speed and Acceleration Limits/2(upSpeedMax)
  zAccMax/1 -> Vertical Speed and Acceleration Limits/3(zAccMax)
  zJerkMax/1 -> Vertical Speed and Acceleration Limits/4(zJerkMax)
  Cutoff Frequency FLTT/1 -> Vertical Speed and Acceleration Limits/6(zAccFltt_f)
  Cutoff Frequency FLTE/1 -> Vertical Speed and Acceleration Limits/7(zAccFlte_f)
  Cutoff Frequency FLTT1/1 -> Vertical Speed and Acceleration Limits/5(GRAVITY_MSS)
  [zVelDes] -> zVelDes/1
  [zVelAct] -> zVelAct/1
  Unit Delay/1 -> [limitThrLower]
  Unit Delay1/1 -> [limitThrUpper]
  inMeas/1 -> Bus Selector/1
  Bus Selector/4 -> Mux1/4  "<zPosTarMeas>"
  Bus Selector/5 -> Mux1/5  "<zVelDesMeas>"
  Bus Selector/7 -> [zAccClkDmod]  "<zAccClkDmod>"
  Bus Selector/6 -> Mux1/6  "<zAccDesMeas>"
  Gain/1 -> Mux/3  "zAccAct"
  zVel/1 -> Gain1/1
  zPos/1 -> Gain2/1
  Bus Selector/1 -> Mux1/1  "<zPosActMeas>"
  Bus Selector/2 -> Mux1/2  "<zVelActMeas>"
  Bus Selector/3 -> Mux1/3  "<zAccActMeas>"
  Mux1/1 -> input handler/2(inMeas)  "inMeas"
  input handler/1(inAct) -> Demux/1
  Mux/1 -> input handler/1(inSim)  "inSim"
  Demux/2 -> [zVelAct]
  Demux/1 -> [zPosAct]
  ctrlInThrottle/1 -> calc des climb rate/1(ctrlIn)
  calc des climb rate/1(climbRate) -> set_pos_target_z_from_climb_rate()/2(climbRateDes)  "climbRateDes"
  [limitThrLower] -> set z component of limit vec/1(limitLower)
  [limitThrUpper] -> set z component of limit vec/2(limitUpper)
  set_pos_target_z_from_climb_rate()/1(posTar) -> Mux/4  "zPosTar"
  set_pos_target_z_from_climb_rate()/2(velDes) -> Mux/5  "zVelDes"
  set_pos_target_z_from_climb_rate()/3(accDes) -> Mux/6  "zAccDes"
  Gain1/1 -> Mux/2  "zVelAct"
  Gain2/1 -> Mux/1  "zPosAct"
  zAcc/1 -> Gain/1
  Demux/3 -> [zAccAct]
  limitThrLower/1 -> Unit Delay/1
  Data Store Read5/1 -> set_pos_target_z_from_climb_rate()/1(posTarIn)
  set z component of limit vec/1(limitVectorZ) -> set_pos_target_z_from_climb_rate()/3(limitVectorZ)
  Data Store Read4/1 -> set_pos_target_z_from_climb_rate()/4(velMaxUp)
  Data Store Read2/1 -> set_pos_target_z_from_climb_rate()/5(velMaxDn)
  Data Store Read1/1 -> set_pos_target_z_from_climb_rate()/6(accMaxZ)
  Data Store Read3/1 -> set_pos_target_z_from_climb_rate()/7(jerkMaxZ)
  P Position z/3(posErr) -> [posErr]
  [velErr] -> Unit Delay2/1
  [posErr] -> Unit Delay3/1
  get_pilot_speed_dn()/1(dnMax) -> Gain3/1
  Gain3/1 -> Vertical Speed and Acceleration Limits/1(dnSpeedMax)
  Unit Delay2/1 -> set_pos_target_z_from_climb_rate()/9(velErr)
  Unit Delay3/1 -> set_pos_target_z_from_climb_rate()/8(posErr)
  Demux/5 -> [zVelDes]
  Demux/6 -> [zAccDes]
  Demux/4 -> [zPosTar]

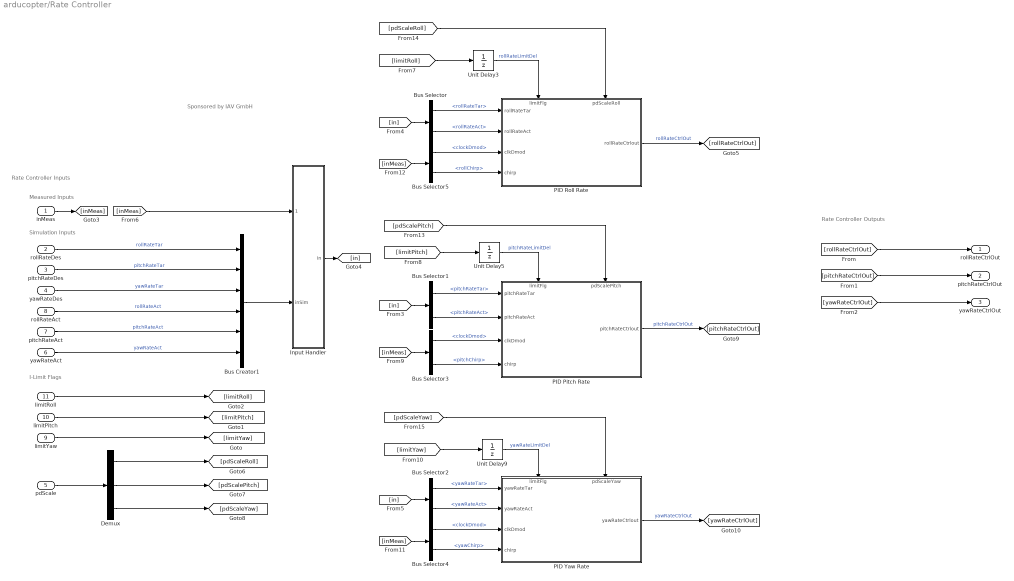
== system arducopter/Rate Controller ==
  note: Rate Controller Inputs
  note: Rate Controller Outputs
  note: I-Limit Flags
  note: Simulation Inputs
  note: Measured Inputs
  note: Sponsored by IAV GmbH
  inMeas : Inport
  rollRateDes : Inport  Port=2
  pitchRateDes : Inport  Port=3
  yawRateDes : Inport  Port=4
  pdScale : Inport  Port=5
  yawRateAct : Inport  Port=6
  pitchRateAct : Inport  Port=7
  rollRateAct : Inport  Port=8
  limitYaw : Inport  Port=9
  limitPitch : Inport  Port=10
  limitRoll : Inport  Port=11
  Bus Creator1 : BusCreator  Inputs=6
  Bus Selector : BusSelector  OutputSignals=rollRateTar,rollRateAct
  Bus Selector1 : BusSelector  OutputSignals=pitchRateTar,pitchRateAct
  Bus Selector2 : BusSelector  OutputSignals=yawRateTar,yawRateAct
  Bus Selector3 : BusSelector  OutputSignals=PIDP.clockDmod,SIDD.mixerChirps.pitchChirp
  Bus Selector4 : BusSelector  OutputSignals=PIDY.clockDmod,SIDD.mixerChirps.yawChirp
  Bus Selector5 : BusSelector  OutputSignals=PIDR.clockDmod,SIDD.mixerChirps.rollChirp
  Demux : Demux  Outputs=3
  Input Handler : Subsystem
  PID Pitch Rate : Subsystem
      settings: PortSchema="{\"entries\":[{\"content\":{\"sides\":[{\"content\":{\"connectorIds\":[\"In1\",\"In2\",\"In3\",\"In4\"]},\"type\":\"ConnectorPlacement.EquallySpacedRectSide\",\"uuid\":\"2a5dbe90-453f-4e9e-99b5-8df933193a67\"},{\"content\":{\"connectorIds\":[\"Out1\"],\"side\":\"RIGHT\"},\"type\":\"ConnectorPlacement.EquallySpacedRectSide\",\"uuid\":\"647d156a-d747-46aa-99b5-4267a31a349a\"},{\"content\":{\"connectorIds\":[\"In5\",\"In6\"],\"side\":\"TOP\"},\"type\":\"ConnectorPlacement.EquallySpacedRectSide\",\"uuid\":\"cd468014-c72e-477d-ab7a-d05ad29c3156\"}]},\"type\":\"ConnectorPlacement.EquallySpacedConnector\",\"uuid\":\"c8588a65-506c-4f80-8a82-377d61761653\"}],\"packageUris\":[\"http://schema.mathworks.com/mf0/Connector/R2020b\"],\"version\":\"1.0\"}"
  PID Roll Rate : Subsystem
      settings: PortSchema="{\"entries\":[{\"content\":{\"sides\":[{\"content\":{\"connectorIds\":[\"In1\",\"In2\",\"In3\",\"In4\"]},\"type\":\"ConnectorPlacement.EquallySpacedRectSide\",\"uuid\":\"e641bc52-3ba8-4abf-91e5-f3e8f1d63eab\"},{\"content\":{\"connectorIds\":[\"Out1\"],\"side\":\"RIGHT\"},\"type\":\"ConnectorPlacement.EquallySpacedRectSide\",\"uuid\":\"7d55638e-b8f2-47ab-a11f-a4e45a3d6a7b\"},{\"content\":{\"connectorIds\":[\"In5\",\"In6\"],\"side\":\"TOP\"},\"type\":\"ConnectorPlacement.EquallySpacedRectSide\",\"uuid\":\"6a487507-9fdf-4d3e-b86b-b3f94c6d2850\"}]},\"type\":\"ConnectorPlacement.EquallySpacedConnector\",\"uuid\":\"38d20622-e21d-450d-bf23-0a2964a9c200\"}],\"packageUris\":[\"http://schema.mathworks.com/mf0/Connector/R2020b\"],\"version\":\"1.0\"}"
  PID Yaw Rate : Subsystem
      settings: PortSchema="{\"entries\":[{\"content\":{\"sides\":[{\"content\":{\"connectorIds\":[\"In1\",\"In2\",\"In3\",\"In4\"]},\"type\":\"ConnectorPlacement.EquallySpacedRectSide\",\"uuid\":\"95e985cf-5aaa-4eec-af88-c33d80501d42\"},{\"content\":{\"connectorIds\":[\"Out1\"],\"side\":\"RIGHT\"},\"type\":\"ConnectorPlacement.EquallySpacedRectSide\",\"uuid\":\"41aa25dd-11fe-476a-b160-e9ff156178ad\"},{\"content\":{\"connectorIds\":[\"In5\",\"In6\"],\"side\":\"TOP\"},\"type\":\"ConnectorPlacement.EquallySpacedRectSide\",\"uuid\":\"b46bb718-16e1-44f9-9a83-d446bf88a339\"}]},\"type\":\"ConnectorPlacement.EquallySpacedConnector\",\"uuid\":\"f9e6c180-8f1d-4955-ab4a-0b277b051f61\"}],\"packageUris\":[\"http://schema.mathworks.com/mf0/Connector/R2020b\"],\"version\":\"1.0\"}"
  Unit Delay3 : UnitDelay  SampleTime=-1  HasFrameUpgradeWarning=on
  Unit Delay5 : UnitDelay  SampleTime=-1  HasFrameUpgradeWarning=on
  Unit Delay9 : UnitDelay  SampleTime=-1  HasFrameUpgradeWarning=on
  rollRateCtrlOut : Outport
  pitchRateCtrlOut : Outport  Port=2
  yawRateCtrlOut : Outport  Port=3
  wires:
  PID Yaw Rate/1(yawRateCtrlout) -> [yawRateCtrlOut]  "yawRateCtrlOut"
  Bus Selector/1 -> PID Roll Rate/1(rollRateTar)  "<rollRateTar>"
  Bus Selector/2 -> PID Roll Rate/2(rollRateAct)  "<rollRateAct>"
  Bus Selector2/1 -> PID Yaw Rate/1(yawRateTar)  "<yawRateTar>"
  [limitYaw] -> Unit Delay9/1
  Unit Delay3/1 -> PID Roll Rate/5(limitFlg)  "rollRateLimitDel"
  [limitRoll] -> Unit Delay3/1
  Bus Selector2/2 -> PID Yaw Rate/2(yawRateAct)  "<yawRateAct>"
  PID Roll Rate/1(rollRateCtrlout) -> [rollRateCtrlOut]  "rollRateCtrlOut"
  [limitPitch] -> Unit Delay5/1
  Unit Delay9/1 -> PID Yaw Rate/5(limitFlg)  "yawRateLimitDel"
  [rollRateCtrlOut] -> rollRateCtrlOut/1
  [pitchRateCtrlOut] -> pitchRateCtrlOut/1
  [yawRateCtrlOut] -> yawRateCtrlOut/1
  limitYaw/1 -> [limitYaw]
  limitPitch/1 -> [limitPitch]
  limitRoll/1 -> [limitRoll]
  rollRateAct/1 -> Bus Creator1/4  "rollRateAct"
  pitchRateAct/1 -> Bus Creator1/5  "pitchRateAct"
  yawRateAct/1 -> Bus Creator1/6  "yawRateAct"
  Bus Creator1/1 -> Input Handler/2(inSim)
  yawRateDes/1 -> Bus Creator1/3  "yawRateTar"
  pitchRateDes/1 -> Bus Creator1/2  "pitchRateTar"
  rollRateDes/1 -> Bus Creator1/1  "rollRateTar"
  Input Handler/1(in) -> [in]
  [in] -> Bus Selector/1
  [in] -> Bus Selector1/1
  [in] -> Bus Selector2/1
  Bus Selector1/1 -> PID Pitch Rate/1(pitchRateTar)  "<pitchRateTar>"
  Bus Selector1/2 -> PID Pitch Rate/2(pitchRateAct)  "<pitchRateAct>"
  inMeas/1 -> [inMeas]
  [inMeas] -> Input Handler/1(inMeas)
  [inMeas] -> Bus Selector3/1
  [inMeas] -> Bus Selector4/1
  Bus Selector4/1 -> PID Yaw Rate/3(clkDmod)  "<clockDmod>"
  Bus Selector4/2 -> PID Yaw Rate/4(chirp)  "<yawChirp>"
  [inMeas] -> Bus Selector5/1
  Bus Selector5/1 -> PID Roll Rate/3(clkDmod)  "<clockDmod>"
  Bus Selector5/2 -> PID Roll Rate/4(chirp)  "<rollChirp>"
  Unit Delay5/1 -> PID Pitch Rate/5(limitFlg)  "pitchRateLimitDel"
  Bus Selector3/2 -> PID Pitch Rate/4(chirp)  "<pitchChirp>"
  pdScale/1 -> Demux/1
  Demux/2 -> [pdScalePitch]
  Demux/1 -> [pdScaleRoll]
  [pdScaleRoll] -> PID Roll Rate/6(pdScaleRoll)
  Bus Selector3/1 -> PID Pitch Rate/3(clkDmod)  "<clockDmod>"
  [pdScalePitch] -> PID Pitch Rate/6(pdScalePitch)
  PID Pitch Rate/1(pitchRateCtrlout) -> [pitchRateCtrlOut]  "pitchRateCtrlOut"
  Demux/3 -> [pdScaleYaw]
  [pdScaleYaw] -> PID Yaw Rate/6(pdScaleYaw)
